simulink model "sfc_6p_6p_topology"  (R2023b)
settings: configuration reference "Configuration" (kept outside this file)
PreLoadFcn:
  | Ts=10e-6;
InitFcn:
  | Ts=10e-6;
values from neighbouring files (symbols this model uses):
  dc_link_inductance = 8e-3    (= 0.008)    [sfc_simulation_parameters.m]
  dc_link_resistance = 0.0503    [sfc_simulation_parameters.m]
  equivalent_grid_side_inductance = 0.4941e-3    (= 0.0004941)    [sfc_simulation_parameters.m]
  equivalent_grid_side_resistance = 0.0163    [sfc_simulation_parameters.m]
  equivalent_machine_side_inductance = 0.2508e-3    (= 0.0002508)    [sfc_simulation_parameters.m]
  equivalent_machine_side_resistance = 0.0066    [sfc_simulation_parameters.m]
libraries: spsControlledVoltageSourceLib x6, spsGroundLib x2, eeGeneralControl x2, spsUniversalBridgeLib x2, spsThreePhaseVIMeasurementLib x2, spsSeriesRLCBranchLib x2, spsThreePhaseSeriesRLCBranchLib x2, spsCurrentMeasurementLib x1, spspowerguiLib x1
settings Model: Creator=The MathWorks, Inc.  LastModifiedBy=CHMABRI9
settings ConfigSetRef: SourceName=Configuration  SourceLocation=Base Workspace

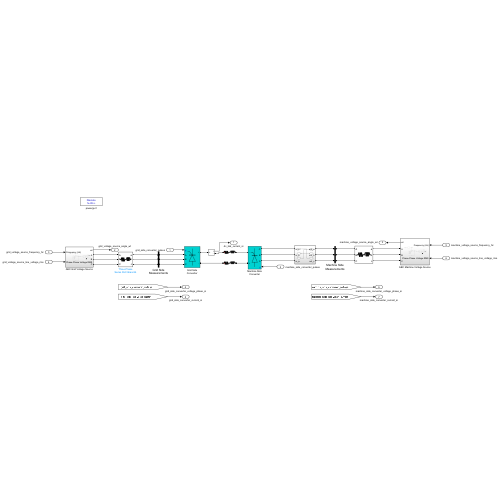
[thumbnail: Simulink's stored preview of the top-level diagram]
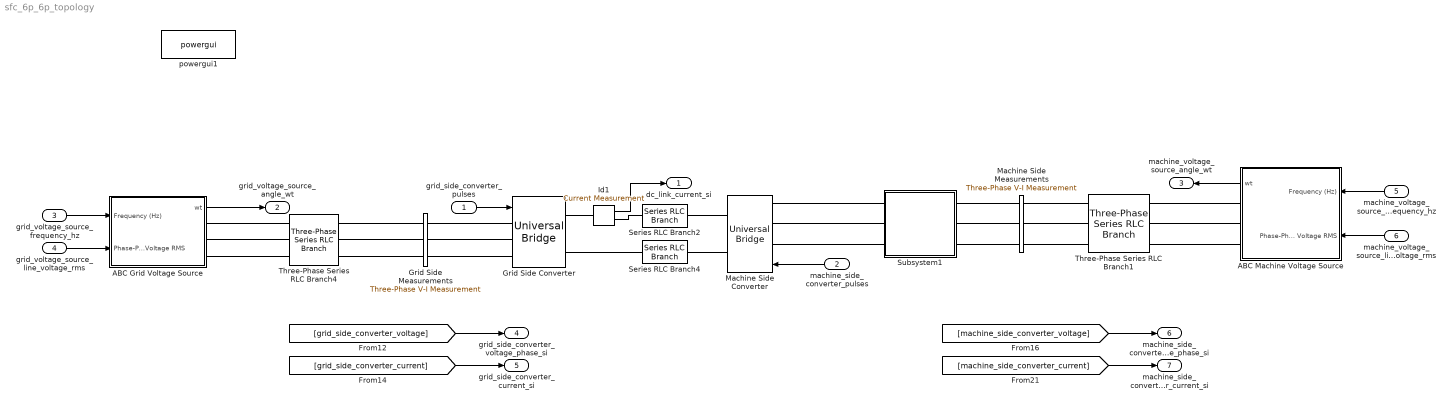
== system sfc_6p_6p_topology ==
  grid_side_converter_pulses : Inport
  machine_side_converter_pulses : Inport  Port=2
  grid_voltage_source_frequency_hz : Inport  Port=3
  grid_voltage_source_line_voltage_rms : Inport  Port=4
  machine_voltage_source_frequency_hz : Inport  Port=5
  machine_voltage_source_line_voltage_rms : Inport  Port=6
  ABC Grid Voltage Source : Subsystem
  ABC Machine Voltage Source : Subsystem
  Grid Side Converter : spsUniversalBridgeLib/Universal Bridge  Arms=3  SnubberResistance=50  SnubberCapacitance=100e-6  Device=Thyristors  Ron=1e-3  Lon=0  ForwardVoltages="[  0  0  ]"  ForwardVoltage=0  GTOparameters=[ 10e-6 , 20e-6 ]  IGBTparameters=[ 1e-6 , 2e-6 ]  Measurements=None  Measurements_2=None  converterType=Rectifier
  Grid Side Measurements : spsThreePhaseVIMeasurementLib/Three-Phase V-I Measurement  VoltageMeasurement=phase-to-ground  SetLabelV=on  LabelV=grid_side_converter_voltage  Vpu=off  VpuLL=off  CurrentMeasurement=yes  SetLabelI=on  LabelI=grid_side_converter_current  Ipu=off  Pbase=100e6  Vbase=2000  OutputType=Complex  PhasorSimulation=off  PSBequivalent=0
  Id1 : spsCurrentMeasurementLib/Current Measurement  Tag=PoWeRsYsTeMmEaSuReMeNt  PhasorSimulation=off  OutputType=Complex  PSBequivalent=0
      settings: AttributesFormatString=\n
  Machine Side Converter : spsUniversalBridgeLib/Universal Bridge  Arms=3  SnubberResistance=50  SnubberCapacitance=100e-6  Device=Thyristors  Ron=1e-3  Lon=0  ForwardVoltages="[  0  0  ]"  ForwardVoltage=0  GTOparameters=[ 10e-6 , 20e-6 ]  IGBTparameters=[ 1e-6 , 2e-6 ]  Measurements=None  Measurements_2=None  converterType=Rectifier
  Machine Side Measurements : spsThreePhaseVIMeasurementLib/Three-Phase V-I Measurement  VoltageMeasurement=phase-to-ground  SetLabelV=on  LabelV=machine_side_converter_voltage  Vpu=off  VpuLL=off  CurrentMeasurement=yes  SetLabelI=on  LabelI=machine_side_converter_current  Ipu=off  Pbase=100e6  Vbase=2000  OutputType=Complex  PhasorSimulation=off  PSBequivalent=0
  Series RLC Branch2 : spsSeriesRLCBranchLib/Series RLC Branch  LConnTagsString=__new0  RConnTagsString=__new0  BranchType=RL  Resistance=dc_link_resistance/2  Inductance=dc_link_inductance/2  SetiL0=off  InitialCurrent=0  Capacitance=[]  Setx0=off  InitialVoltage=0  Measurements=Branch current
  Series RLC Branch4 : spsSeriesRLCBranchLib/Series RLC Branch  LConnTagsString=__new0  RConnTagsString=__new0  BranchType=RL  Resistance=dc_link_resistance/2  Inductance=dc_link_inductance/2  SetiL0=off  InitialCurrent=0  Capacitance=[]  Setx0=off  InitialVoltage=0  Measurements=None
  Subsystem1 : Subsystem
  Three-Phase Series RLC Branch1 : spsThreePhaseSeriesRLCBranchLib/Three-Phase Series RLC Branch  LConnTagsString=A|B|C  RConnTagsString=A|B|C  BranchType=RL  Resistance=equivalent_machine_side_resistance  Inductance=equivalent_machine_side_inductance  Capacitance=0  Measurements=None
  Three-Phase Series RLC Branch4 : spsThreePhaseSeriesRLCBranchLib/Three-Phase Series RLC Branch  LConnTagsString=A|B|C  RConnTagsString=A|B|C  BranchType=RL  Resistance=equivalent_grid_side_resistance  Inductance=equivalent_grid_side_inductance  Capacitance=0  Measurements=None
  powergui1 : spspowerguiLib/powergui  Priority=1  SimulationMode=Discrete  SampleTime=10e-6  frequency=60  Iterations=50  frequencyindice=0  Pbase=100e6  ErrMax=0.0001  UnitsV=kV  UnitsW=MW  buscounter=0  FunctionMessages=off  echomessages=off  EnableUseOfTLC=off  CurrentSourceSwitches=off  DisableSnubberDevices=on  DisableRonSwitches=on  DisableVfSwitches=on  DisplayEquations=off  AutomaticDiscreteSolvers=off  SolverType=Tustin/Backward Euler (TBE)  Interpol=off  ExternalGateDelay=off  methode=off  Ts=100  x0status=blocks  SPID=on  SwTol=0  HookPort=off  NonlinearTolerance=1e-4  nMaxIteration=100  ContinueOnMaxIteration=off  RestoreLinks=warning  ResistiveCurrentMeasurement=off  Frange=[0:2:500]  Ylog=off  Xlog=on  ShowGrid=off  save=off  variable=ZData  structure=ScopeData1  ZoomFFT=off  StartTime=0.08-2/60  cycles=2  DisplayStyle=1  fundamental=60  FreqAxis=on  MaxFrequency=2000  frequencyindicesteady=1  RmsSteady=1  display=off
  dc_link_current_si : Outport
  grid_voltage_source_angle_wt : Outport  Port=2
  machine_voltage_source_angle_wt : Outport  Port=3
  grid_side_converter_voltage_phase_si : Outport  Port=4
  grid_side_converter_current_si : Outport  Port=5
  machine_side_converter_voltage_phase_si : Outport  Port=6
  machine_side_converter_current_si : Outport  Port=7
  wires:
  ABC Grid Voltage Source/1(wt) -> grid_voltage_source_angle_wt/1
  grid_side_converter_pulses/1 -> Grid Side Converter/1
  ABC Machine Voltage Source/1(wt) -> machine_voltage_source_angle_wt/1
  grid_voltage_source_frequency_hz/1 -> ABC Grid Voltage Source/1(Frequency (Hz))
  Id1/1 -> dc_link_current_si/1
  machine_voltage_source_line_voltage_rms/1 -> ABC Machine Voltage Source/2(Phase-Phase Voltage RMS)
  machine_side_converter_pulses/1 -> Machine Side Converter/1
  [grid_side_converter_voltage] -> grid_side_converter_voltage_phase_si/1
  [machine_side_converter_current] -> machine_side_converter_current_si/1
  [grid_side_converter_current] -> grid_side_converter_current_si/1
  machine_voltage_source_frequency_hz/1 -> ABC Machine Voltage Source/1(Frequency (Hz))
  [machine_side_converter_voltage] -> machine_side_converter_voltage_phase_si/1
  grid_voltage_source_line_voltage_rms/1 -> ABC Grid Voltage Source/2(Phase-Phase Voltage RMS)
  connections:
  Three-Phase Series RLC Branch1/RConn3 -- ABC Machine Voltage Source/RConn3
  Three-Phase Series RLC Branch1/LConn1 -- Machine Side Measurements/RConn1
  Subsystem1/LConn2 -- Machine Side Converter/LConn2
  Machine Side Measurements/LConn2 -- Subsystem1/RConn2
  Subsystem1/RConn3 -- Machine Side Measurements/LConn3
  Subsystem1/RConn1 -- Machine Side Measurements/LConn1
  Series RLC Branch4/RConn1 -- Machine Side Converter/RConn1
  Three-Phase Series RLC Branch1/LConn3 -- Machine Side Measurements/RConn3
  Three-Phase Series RLC Branch4/RConn2 -- Grid Side Measurements/LConn2
  Grid Side Measurements/RConn3 -- Grid Side Converter/LConn3
  Three-Phase Series RLC Branch1/RConn2 -- ABC Machine Voltage Source/RConn2
  Series RLC Branch2/LConn1 -- Id1/RConn1
  Subsystem1/LConn1 -- Machine Side Converter/LConn3
  Grid Side Measurements/RConn1 -- Grid Side Converter/LConn1
  Grid Side Converter/LConn2 -- Grid Side Measurements/RConn2
  Series RLC Branch4/LConn1 -- Grid Side Converter/RConn2
  Subsystem1/LConn3 -- Machine Side Converter/LConn1
  Three-Phase Series RLC Branch4/RConn3 -- Grid Side Measurements/LConn3
  Three-Phase Series RLC Branch4/LConn3 -- ABC Grid Voltage Source/RConn3
  Three-Phase Series RLC Branch1/RConn1 -- ABC Machine Voltage Source/RConn1
  Three-Phase Series RLC Branch4/LConn2 -- ABC Grid Voltage Source/RConn2
  Three-Phase Series RLC Branch4/LConn1 -- ABC Grid Voltage Source/RConn1
  Three-Phase Series RLC Branch1/LConn2 -- Machine Side Measurements/RConn2
  Series RLC Branch2/RConn1 -- Machine Side Converter/RConn2
  Id1/LConn1 -- Grid Side Converter/RConn1
  Three-Phase Series RLC Branch4/RConn1 -- Grid Side Measurements/LConn1

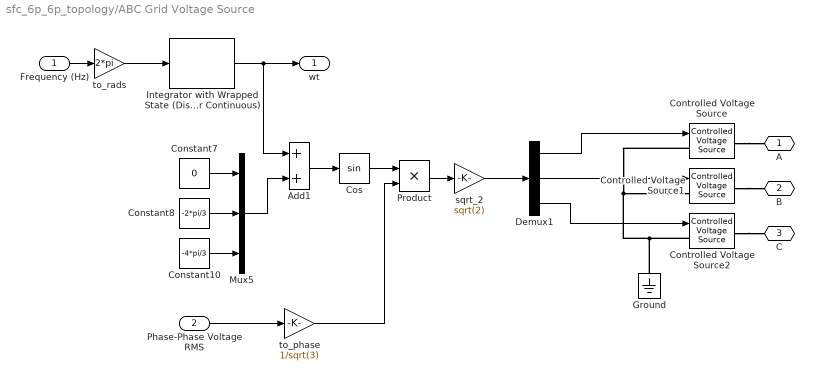
== system sfc_6p_6p_topology/ABC Grid Voltage Source ==
  Frequency (Hz) : Inport
  Phase-Phase Voltage RMS : Inport  Port=2
  Add1 : Sum
  Constant10 : Constant  Value=-4*pi/3
  Constant7 : Constant  Value=0
  Constant8 : Constant  Value=-2*pi/3
  Controlled Voltage Source : spsControlledVoltageSourceLib/Controlled Voltage Source  Initialize=on  Source_Type=AC  Amplitude=0  Phase=0  Frequency=0  Measurements=None
  Controlled Voltage Source1 : spsControlledVoltageSourceLib/Controlled Voltage Source  Initialize=on  Source_Type=AC  Amplitude=0  Phase=0  Frequency=0  Measurements=None
  Controlled Voltage Source2 : spsControlledVoltageSourceLib/Controlled Voltage Source  Initialize=on  Source_Type=AC  Amplitude=0  Phase=0  Frequency=0  Measurements=None
  Cos : Trigonometry
  Demux1 : Demux  Outputs=3
  Ground : spsGroundLib/Ground  LConnTagsString=a
  Integrator with Wrapped State (Discrete or Continuous) : eeGeneralControl/Integrator with Wrapped State (Discrete or Continuous)  LabelModeActiveChoice=Discrete  WrappedStateUpperValue=2*pi  WrappedStateLowerValue=0  x0=0  Ts=-1
      settings: LibrarySourceBlock=|
      | ee_sl_lib/General Control/Integrator with
      | Wrapped State
      | (Discrete or Continuous)
  Mux5 : Mux  Inputs=3
  Product : Product
  sqrt_2 : Gain  Gain=sqrt(2)
  to_phase : Gain  Gain=1/sqrt(3)
  to_rads : Gain  Gain=2*pi
  A : PMIOPort  Side=Right
  B : PMIOPort  Port=2  Side=Right
  C : PMIOPort  Port=3  Side=Right
  wt : Outport
  wires:
  Frequency (Hz)/1 -> to_rads/1
  Mux5/1 -> Add1/2
  Constant8/1 -> Mux5/2
  Demux1/3 -> Controlled Voltage Source2/1
  Demux1/1 -> Controlled Voltage Source/1
  Integrator with Wrapped State (Discrete or Continuous)/1 -> Add1/1, wt/1
  Constant10/1 -> Mux5/3
  Demux1/2 -> Controlled Voltage Source1/1
  Add1/1 -> Cos/1
  Constant7/1 -> Mux5/1
  Cos/1 -> Product/1
  Product/1 -> sqrt_2/1
  sqrt_2/1 -> Demux1/1
  Phase-Phase Voltage RMS/1 -> to_phase/1
  to_rads/1 -> Integrator with Wrapped State (Discrete or Continuous)/1
  to_phase/1 -> Product/2
  connections:
  Controlled Voltage Source/LConn1 -- Ground/LConn1 -- Controlled Voltage Source2/LConn1 -- Controlled Voltage Source1/LConn1
  Controlled Voltage Source2/RConn1 -- C/RConn1
  Controlled Voltage Source/RConn1 -- A/RConn1
  Controlled Voltage Source1/RConn1 -- B/RConn1

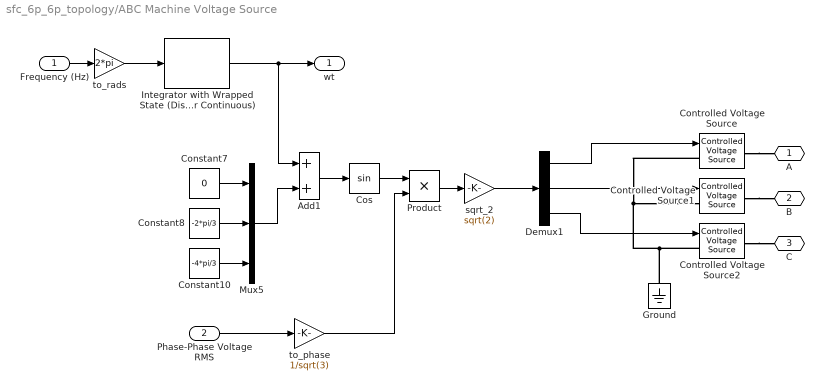
== system sfc_6p_6p_topology/ABC Machine Voltage Source ==
  Frequency (Hz) : Inport
  Phase-Phase Voltage RMS : Inport  Port=2
  Add1 : Sum
  Constant10 : Constant  Value=-4*pi/3
  Constant7 : Constant  Value=0
  Constant8 : Constant  Value=-2*pi/3
  Controlled Voltage Source : spsControlledVoltageSourceLib/Controlled Voltage Source  Initialize=on  Source_Type=AC  Amplitude=0  Phase=0  Frequency=0  Measurements=None
  Controlled Voltage Source1 : spsControlledVoltageSourceLib/Controlled Voltage Source  Initialize=on  Source_Type=AC  Amplitude=0  Phase=0  Frequency=0  Measurements=None
  Controlled Voltage Source2 : spsControlledVoltageSourceLib/Controlled Voltage Source  Initialize=on  Source_Type=AC  Amplitude=0  Phase=0  Frequency=0  Measurements=None
  Cos : Trigonometry
  Demux1 : Demux  Outputs=3
  Ground : spsGroundLib/Ground  LConnTagsString=a
  Integrator with Wrapped State (Discrete or Continuous) : eeGeneralControl/Integrator with Wrapped State (Discrete or Continuous)  LabelModeActiveChoice=Discrete  WrappedStateUpperValue=2*pi  WrappedStateLowerValue=0  x0=0  Ts=-1
      settings: LibrarySourceBlock=|
      | ee_sl_lib/General Control/Integrator with
      | Wrapped State
      | (Discrete or Continuous)
  Mux5 : Mux  Inputs=3
  Product : Product
  sqrt_2 : Gain  Gain=sqrt(2)
  to_phase : Gain  Gain=1/sqrt(3)
  to_rads : Gain  Gain=2*pi
  A : PMIOPort  Side=Right
  B : PMIOPort  Port=2  Side=Right
  C : PMIOPort  Port=3  Side=Right
  wt : Outport
  wires:
  Frequency (Hz)/1 -> to_rads/1
  Mux5/1 -> Add1/2
  Constant8/1 -> Mux5/2
  Demux1/3 -> Controlled Voltage Source2/1
  Demux1/1 -> Controlled Voltage Source/1
  Integrator with Wrapped State (Discrete or Continuous)/1 -> Add1/1, wt/1
  Constant10/1 -> Mux5/3
  Demux1/2 -> Controlled Voltage Source1/1
  Add1/1 -> Cos/1
  Constant7/1 -> Mux5/1
  Cos/1 -> Product/1
  Product/1 -> sqrt_2/1
  sqrt_2/1 -> Demux1/1
  Phase-Phase Voltage RMS/1 -> to_phase/1
  to_rads/1 -> Integrator with Wrapped State (Discrete or Continuous)/1
  to_phase/1 -> Product/2
  connections:
  Controlled Voltage Source1/LConn1 -- Controlled Voltage Source/LConn1 -- Controlled Voltage Source2/LConn1 -- Ground/LConn1
  Controlled Voltage Source2/RConn1 -- C/RConn1
  Controlled Voltage Source/RConn1 -- A/RConn1
  Controlled Voltage Source1/RConn1 -- B/RConn1

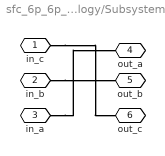
== system sfc_6p_6p_topology/Subsystem1 ==
  in_c : PMIOPort  Side=Left
  in_b : PMIOPort  Port=2  Side=Left
  in_a : PMIOPort  Port=3  Side=Left
  out_a : PMIOPort  Port=4  Side=Right
  out_b : PMIOPort  Port=5  Side=Right
  out_c : PMIOPort  Port=6  Side=Right
  connections:
  in_a/RConn1 -- out_a/RConn1
  in_c/RConn1 -- out_c/RConn1
  in_b/RConn1 -- out_b/RConn1
